simulink model "base"  (R2025a)
settings: Solver=VariableStepAuto  StartTime=10  StopTime=24  RelTol=1e-3
undefined symbols (not defined in the file): DiscIntNeverNeededParam
libraries: spsSeriesRLCBranchLib x4, spsGroundLib x3, spsVoltageMeasurementLib x3, spsCurrentMeasurementLib x2, powerlib_extras x2, spsControlledVoltageSourceLib x1, fuzblock x1, spsDiodeLib x1, spsMosfetLib x1, spsPVArrayLib x1, spsPWMGenerator2LevelLib x1, sps_lib x1
settings Model: Creator=Rishitha  LastModifiedBy=Rishitha

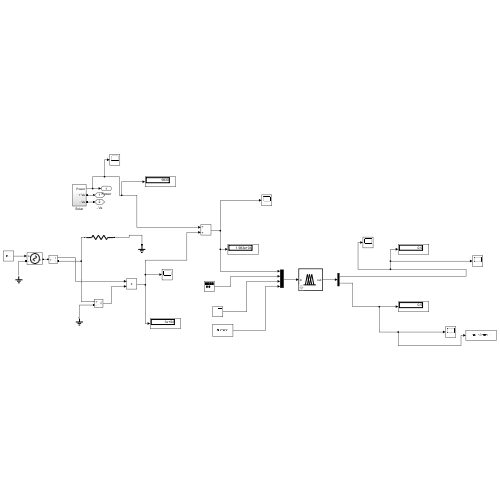
[thumbnail: Simulink's stored preview of the top-level diagram]
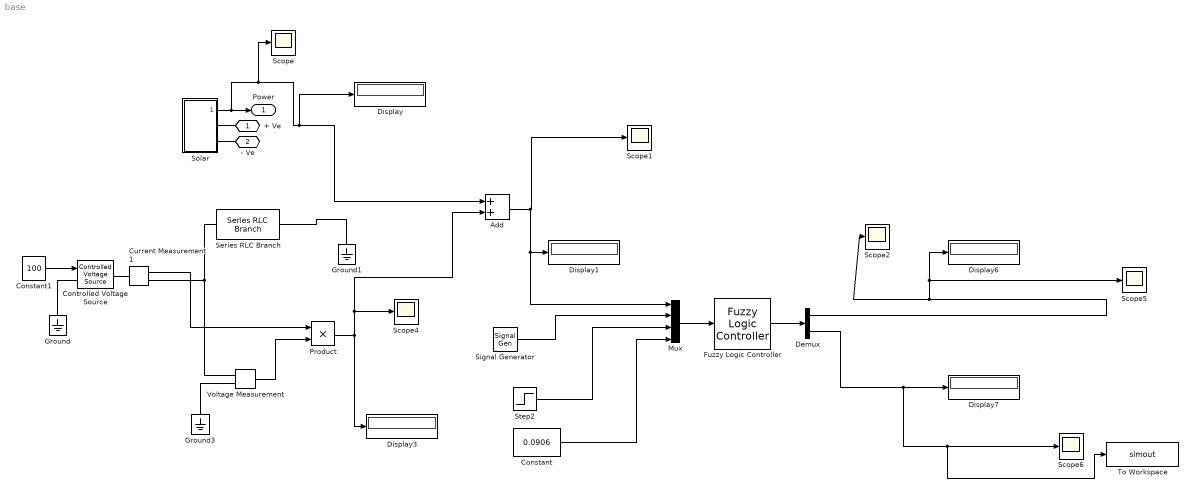
== system base ==
  Add : Sum
  Constant : Constant  Value=0.0906
  Constant1 : Constant  Value=100
  Controlled Voltage Source : spsControlledVoltageSourceLib/Controlled Voltage Source  Initialize=on  Source_Type=AC  Amplitude=0  Phase=0  Frequency=0  Measurements=None
  Current Measurement1 : spsCurrentMeasurementLib/Current Measurement  PhasorSimulation=off  OutputType=Complex  PSBequivalent=0
  Demux : Demux  Outputs=2
  Display{,1,3,6..7} (5 alike) : Display
  Fuzzy Logic Controller : fuzblock/Fuzzy Logic  Controller  FIS="\"C:\\SEM-5\\Control Systems\\Project\\evcs_fuzzy.fis\""  OutputSampleNumber=101  DataType=double  UseLookupTable=on  NumBreakpoints=4  FuzzifiedInputs=off  RuleFiringStrengths=off  RuleOutputs=off  AggregatedOutputs=off  SimulateUsing=Interpreted execution  OutOfRangeInputValueMessage=warning  NoRuleFiredMessage=warning  EmptyOutputFuzzySetMessage=warning
  Ground : spsGroundLib/Ground  LConnTagsString=a
  Ground1 : spsGroundLib/Ground  LConnTagsString=a
  Ground3 : spsGroundLib/Ground  LConnTagsString=a
  Mux : Mux
  Product : Product
  Scope{,1..2,4..6} (6 alike) : Scope
      Scope1 settings: DataLoggingVariableName=ScopeData9
      Scope2 settings: ActiveDisplayYMinimum=0.7644094488188975  ActiveDisplayYMaximum=0.96440944881889745  DataLoggingVariableName=ScopeData10
      Scope4 settings: ActiveDisplayYMinimum=9000  ActiveDisplayYMaximum=11000  DataLoggingVariableName=ScopeData12
      Scope5 settings: ActiveDisplayYMinimum=0.45444881889763783  ActiveDisplayYMaximum=0.9099606299212597  DataLoggingVariableName=ScopeData13
      Scope6 settings: ActiveDisplayYMinimum=0.456153969658102  ActiveDisplayYMaximum=0.8946142730770823  DataLoggingVariableName=ScopeData14
  Series RLC Branch : spsSeriesRLCBranchLib/Series RLC Branch  LConnTagsString=__new0  RConnTagsString=__new0  BranchType=R  Resistance=1  Inductance=1e-3  SetiL0=off  InitialCurrent=0  Capacitance=1e-6  Setx0=off  InitialVoltage=0  Measurements=None
  Signal Generator : SignalGenerator  Units=rad/sec
  Solar : Subsystem
  Step2 : Step  Time=17  SampleTime=0
  To Workspace : ToWorkspace  VariableName=simout  SaveFormat=Timeseries  SampleTime=-1
  Voltage Measurement : spsVoltageMeasurementLib/Voltage Measurement  PhasorSimulation=off  OutputType=Complex  PSBequivalent=0
  + Ve : PMIOPort  Side=Right
  - Ve : PMIOPort  Port=2  Side=Right
  Power : Outport  VectorParamsAs1DForOutWhenUnconnected=off
  wires:
  Solar/1(Power) -> Add/1, Display/1, Scope/1, Power/1
  Add/1 -> Scope1/1, Mux/1, Display1/1
  Constant/1 -> Mux/4
  Step2/1 -> Mux/3
  Mux/1 -> Fuzzy Logic Controller/1
  Signal Generator/1 -> Mux/2
  Fuzzy Logic Controller/1 -> Demux/1
  Demux/1 -> Display6/1, Scope5/1, Scope2/1
  Demux/2 -> To Workspace/1, Scope6/1, Display7/1
  Voltage Measurement/1 -> Product/2
  Constant1/1 -> Controlled Voltage Source/1
  Product/1 -> Scope4/1, Add/2, Display3/1
  Current Measurement1/1 -> Product/1
  connections:
  Solar/RConn1 -- + Ve/RConn1
  Solar/RConn2 -- - Ve/RConn1
  Voltage Measurement/LConn1 -- Series RLC Branch/LConn1 -- Current Measurement1/RConn1
  Voltage Measurement/LConn2 -- Ground3/LConn1
  Controlled Voltage Source/LConn1 -- Ground/LConn1
  Series RLC Branch/RConn1 -- Ground1/LConn1
  Controlled Voltage Source/RConn1 -- Current Measurement1/LConn1

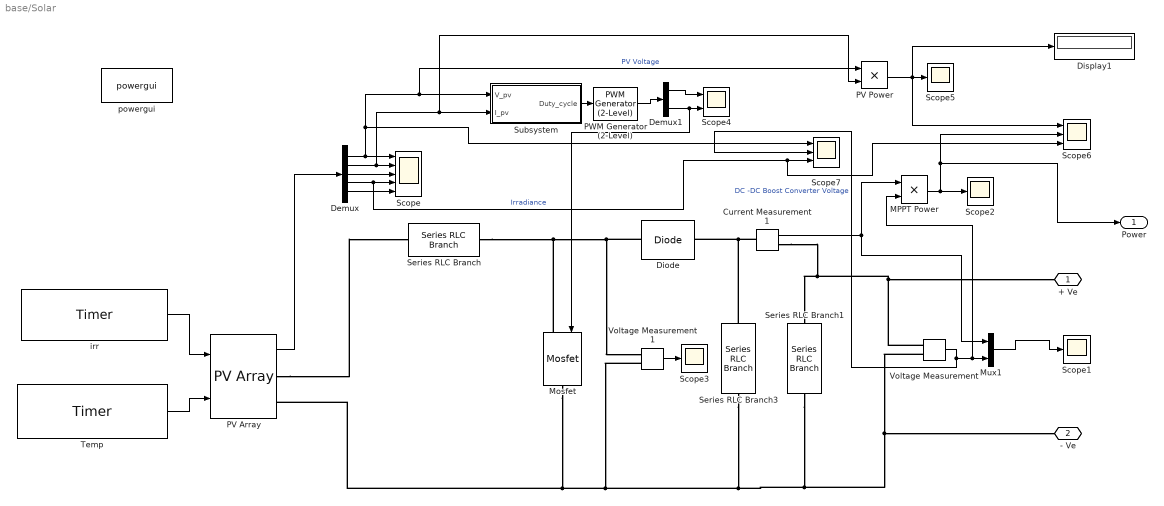
== system base/Solar ==
  Current Measurement1 : spsCurrentMeasurementLib/Current Measurement  PhasorSimulation=off  OutputType=Complex  PSBequivalent=0
  Demux : Demux  Outputs=5
  Demux1 : Demux  Outputs=2
  Diode : spsDiodeLib/Diode  Ron=0.5  Lon=0  Vf=0.7  IC=0  UseSnubber=0  Rs=1e5  Cs=250e-9  Measurements=off
  Display1 : Display
  MPPT Power : Product
  Mosfet : spsMosfetLib/Mosfet  Ron=0.1  Lon=0  Rd=0.01  Vfd=0.7  IC=0  Rs=1e5  Cs=inf  Measurements=off
  Mux1 : Mux  Inputs=2
  PV Array : spsPVArrayLib/PV Array  Npar=15  Nser=10  PlotType=array @ 1000 W/m2 & specified temperatures  S_vec="[ 1000  500  100 ]"  Temp_C_vec="[ 45 25  ]"  ModuleName=User-defined  PlotWhenSelected=off  Pm=213.15  Ncell=60  Voc=36.3  Isc=7.84  Vm=29  Im=7.35  beta_Voc_pc=-0.36099  alpha_Isc_pc=0.102  beta_Voc=-0.13104  alpha_Isc=0.0079968  IL=7.8654  I0=2.9273e-10  nI=0.98119  Rsh=313.0553  Rs=0.39381  RobustModel=off  RobustCellTemperature=313.3991  BAL=off  Tc=1e-6  Tfilter=5e-5
  PV Power : Product
  PWM Generator (2-Level) : spsPWMGenerator2LevelLib/PWM Generator (2-Level)  ModulatorType=Single-phase half-bridge (2 pulses)  ModulatorMode=Unsynchronized  Fc=5000  Pc=0  nF=27  MinMax="[ 0  1 ]"  SamplingTechnique=Natural  ModulatingSignals=off  m=0.8  Freq=60  Phase=0  Ts=0  ShowCarrierOutport=off
  Scope : Scope  NumInputPorts=5
      settings: ActiveDisplayYMinimum=33.56899  ActiveDisplayYMaximum=396.03805
  Scope{1..3,5} (4 alike) : Scope
      Scope1 settings: Title=Fuzzy  ActiveDisplayYMinimum=-62.75545  ActiveDisplayYMaximum=587.88515  DataLoggingVariableName=ScopeData2
      Scope2 settings: ActiveDisplayYMinimum=-1  ActiveDisplayYMaximum=1  DataLoggingVariableName=ScopeData3
      Scope3 settings: ActiveDisplayYMinimum=-67.82899  ActiveDisplayYMaximum=630.78639  DataLoggingVariableName=ScopeData4
      Scope5 settings: ActiveDisplayYMinimum=-1  ActiveDisplayYMaximum=1  DataLoggingVariableName=ScopeData6
  Scope4 : Scope  NumInputPorts=2
      settings: ActiveDisplayYMinimum=-0.125  ActiveDisplayYMaximum=1.125  DataLoggingVariableName=ScopeData5
  Scope6 : Scope  NumInputPorts=3
      settings: Title=PV Output Power  ActiveDisplayYMinimum=-1  ActiveDisplayYMaximum=1  YLabel=Watts  DataLoggingVariableName=ScopeData7
  Scope7 : Scope  NumInputPorts=3
      settings: ActiveDisplayYMinimum=35.55743  ActiveDisplayYMaximum=365.47852  YLabel=voltage  DataLoggingVariableName=ScopeData8
  Series RLC Branch : spsSeriesRLCBranchLib/Series RLC Branch  LConnTagsString=__new0  RConnTagsString=__new0  BranchType=L  Resistance=0.001  Inductance=740e-6  SetiL0=off  InitialCurrent=0  Capacitance=1e-6  Setx0=off  InitialVoltage=0  Measurements=None
  Series RLC Branch1 : spsSeriesRLCBranchLib/Series RLC Branch  LConnTagsString=__new0  RConnTagsString=__new0  BranchType=R  Resistance=10.5  Inductance=0.1  SetiL0=off  InitialCurrent=0  Capacitance=100e-6  Setx0=off  InitialVoltage=0  Measurements=None
  Series RLC Branch3 : spsSeriesRLCBranchLib/Series RLC Branch  LConnTagsString=__new0  RConnTagsString=__new0  BranchType=C  Resistance=6  Inductance=0.1  SetiL0=off  InitialCurrent=0  Capacitance=1100e-6  Setx0=off  InitialVoltage=0  Measurements=None
  Subsystem : Subsystem
  Temp : powerlib_extras/Control  Blocks/Timer  t=[0 .1 .2 .3 .4 .5 .6 .7 .8 .9 1 ]  e=[20 23 25 25 26 27 28 25 24 22 22]
  Voltage Measurement : spsVoltageMeasurementLib/Voltage Measurement  PhasorSimulation=off  OutputType=Complex  PSBequivalent=0
  Voltage Measurement1 : spsVoltageMeasurementLib/Voltage Measurement  PhasorSimulation=off  OutputType=Complex  PSBequivalent=0
  "irr " : powerlib_extras/Control  Blocks/Timer  t=[0 0.049 0.05 0.1 .15 .2 .25 .3 .35 0.4 .45 .5 .6 .7 .8 0.9 1]  e=[0 0 250 400 500 600 700 800 1000 1000 1000 900 800 700 300 100 500]
  powergui : sps_lib/powergui  Priority=1  SimulationMode=Discrete  SampleTime=1e-3  frequency=60  Iterations=50  frequencyindice=0  Pbase=100e6  ErrMax=1e-4  UnitsV=kV  UnitsW=MW  buscounter=0  FunctionMessages=off  echomessages=off  EnableUseOfTLC=off  CurrentSourceSwitches=off  DisableSnubberDevices=off  DisableRonSwitches=off  DisableVfSwitches=off  DisplayEquations=off  AutomaticDiscreteSolvers=off  SolverType=Tustin/Backward Euler (TBE)  Interpol=off  ExternalGateDelay=off  methode=off  Ts=100  x0status=blocks  SPID=on  SwTol=0  HookPort=off  NonlinearTolerance=1e-4  nMaxIteration=100  ContinueOnMaxIteration=off  RestoreLinks=warning  ResistiveCurrentMeasurement=off  Frange=[0:2:500]  Ylog=off  Xlog=on  ShowGrid=off  save=off  variable=ZData  structure=0  ZoomFFT=off  StartTime=0.0  cycles=1  DisplayStyle=1  fundamental=60  FreqAxis=off  MaxFrequency=1000  frequencyindicesteady=1  RmsSteady=1  display=off
  + Ve : PMIOPort  Side=Right
  - Ve : PMIOPort  Port=2  Side=Right
  Power : Outport  VectorParamsAs1DForOutWhenUnconnected=off
  wires:
  PV Power/1 -> Scope6/1, Display1/1, Scope5/1
  Voltage Measurement/1 -> MPPT Power/2, Mux1/2, Scope7/2  "DC -DC Boost Converter Voltage"
  Current Measurement1/1 -> MPPT Power/1, Mux1/1
  MPPT Power/1 -> Power/1, Scope6/2, Scope2/1
  Demux/2 -> Subsystem/2(I_pv), PV Power/2, Scope/2
  Demux1/2 -> Mosfet/1, Scope4/2
  Demux1/1 -> Scope4/1
  "irr "/1 -> PV Array/1
  Voltage Measurement1/1 -> Scope3/1
  Demux/3 -> Scope/3
  PWM Generator (2-Level)/1 -> Demux1/1
  Demux/1 -> Scope7/1, Subsystem/1(V_pv), PV Power/1, Scope/1  "PV Voltage"
  Mux1/1 -> Scope1/1
  Demux/4 -> Scope6/3, Scope7/3, Scope/4  "Irradiance"
  Temp/1 -> PV Array/2
  Subsystem/1(Duty_cycle) -> PWM Generator (2-Level)/1
  Demux/5 -> Scope/5
  PV Array/1 -> Demux/1
  connections:
  Diode/LConn1 -- Mosfet/LConn1 -- Series RLC Branch/RConn1 -- Voltage Measurement1/LConn1
  PV Array/RConn2 -- - Ve/RConn1 -- Voltage Measurement/LConn2 -- Series RLC Branch1/RConn1 -- Series RLC Branch3/RConn1 -- Voltage Measurement1/LConn2 -- Mosfet/RConn1
  Current Measurement1/RConn1 -- Series RLC Branch1/LConn1 -- + Ve/RConn1 -- Voltage Measurement/LConn1
  Current Measurement1/LConn1 -- Series RLC Branch3/LConn1 -- Diode/RConn1
  PV Array/RConn1 -- Series RLC Branch/LConn1

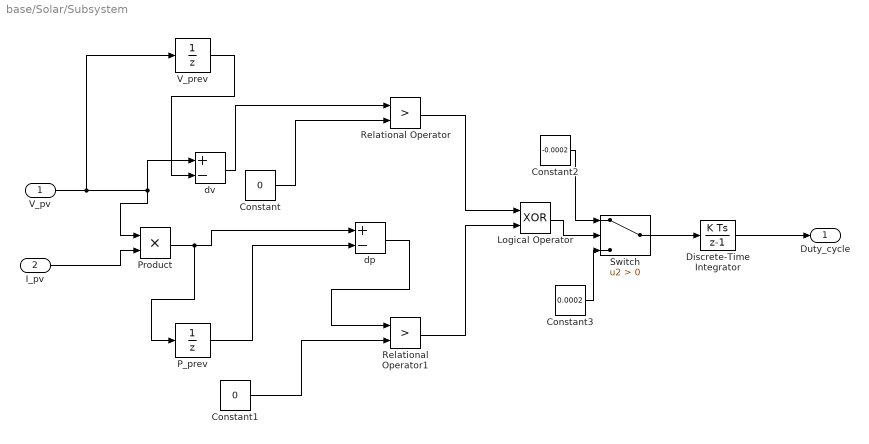
== system base/Solar/Subsystem ==
  V_pv : Inport
  I_pv : Inport  Port=2
  Constant : Constant  Value=0
  Constant1 : Constant  Value=0
  Constant2 : Constant  Value=-0.0002
  Constant3 : Constant  Value=0.0002
  Discrete-Time Integrator : DiscreteIntegrator  InitialCondition=0.5  SampleTime=1e-3  LimitOutput=on  UpperSaturationLimit=1  LowerSaturationLimit=0  ICPrevOutput=DiscIntNeverNeededParam  ICPrevScaledInput=DiscIntNeverNeededParam
  Logical Operator : Logic  Operator=XOR  AllPortsSameDT=off  OutDataTypeStr=boolean
  P_prev : UnitDelay  SampleTime=-1  HasFrameUpgradeWarning=on
  Product : Product
  Relational Operator : RelationalOperator  Operator=>  OutDataTypeStr=boolean  RndMeth=Simplest  InputSameDT=off
  Relational Operator1 : RelationalOperator  Operator=>  OutDataTypeStr=boolean  RndMeth=Simplest  InputSameDT=off
  Switch : Switch  Criteria=u2 > Threshold  SaturateOnIntegerOverflow=off  InputSameDT=off
  V_prev : UnitDelay  SampleTime=-1  HasFrameUpgradeWarning=on
  dp : Sum  Inputs=+-
  dv : Sum  Inputs=+-
  Duty_cycle : Outport
  wires:
  V_pv/1 -> Product/1, dv/1, V_prev/1
  I_pv/1 -> Product/2
  Product/1 -> dp/1, P_prev/1
  P_prev/1 -> dp/2
  V_prev/1 -> dv/2
  dv/1 -> Relational Operator/1
  dp/1 -> Relational Operator1/1
  Constant/1 -> Relational Operator/2
  Constant1/1 -> Relational Operator1/2
  Relational Operator/1 -> Logical Operator/1
  Relational Operator1/1 -> Logical Operator/2
  Logical Operator/1 -> Switch/2
  Constant2/1 -> Switch/1
  Constant3/1 -> Switch/3
  Switch/1 -> Discrete-Time Integrator/1
  Discrete-Time Integrator/1 -> Duty_cycle/1
